simulink model "PUMA_Dynamicssoal4"  (R2026a)
settings: Solver=ode45  StopTime=15  EnableMultiTasking=on
settings Model: Creator=imi-pc
settings DataIOCC: SaveFormat=StructureWithTime
settings HardwareCC: ProdHWDeviceType=Specified
settings GRTTargetCC: CombineOutputUpdateFcns=off  GRTInterface=on

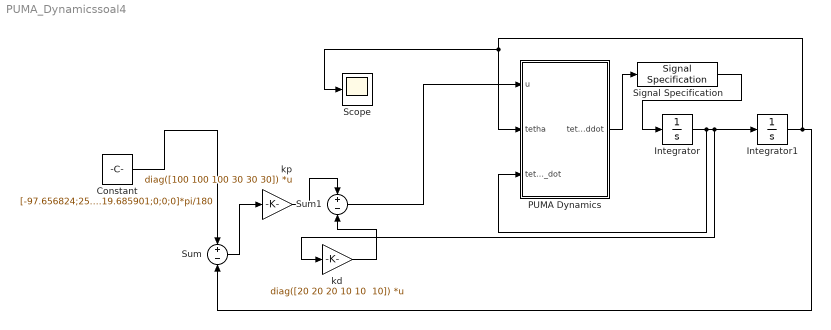
== system PUMA_Dynamicssoal4 ==
  Constant : Constant  Value=[-97.656824;25.988513;-19.685901;0;0;0]*pi/180
  Integrator : Integrator
  Integrator1 : Integrator
  PUMA Dynamics : MATLAB Function  TreatAsAtomicUnit=on
  Scope : Scope
      settings: ActiveDisplayYMinimum=-15.492496269263574  ActiveDisplayYMaximum=5.656821021719038
  Signal Specification : SignalSpecification  Dimensions=[6 1]
  Sum : Sum  Inputs=+-
  Sum1 : Sum  Inputs=+-
  kd : Gain  Gain="diag([20 20 20 10 10  10])"  Multiplication=Matrix(K*u)
  kp : Gain  Gain=diag([100 100 100 30 30 30])  Multiplication=Matrix(K*u)
  wires:
  Integrator/1 -> PUMA Dynamics/3(tetha_dot), kd/1, Integrator1/1
  Constant/1 -> Sum/1
  Sum/1 -> kp/1
  kd/1 -> Sum1/2
  kp/1 -> Sum1/1
  Sum1/1 -> PUMA Dynamics/1(u)
  PUMA Dynamics/1(tetha_ddot) -> Signal Specification/1
  Signal Specification/1 -> Integrator/1
  Integrator1/1 -> Scope/1, PUMA Dynamics/2(tetha), Sum/2

== matlab function PUMA_Dynamicssoal4/PUMA Dynamics ==
  data: u input; tetha input; tetha_ddot output; tetha_dot input
function tetha_ddot = fcn(u,tetha,tetha_dot)






c2=cos(tetha(2));
s2=sin(tetha(2));

c3=cos(tetha(3));
s3=sin(tetha(3));

c23=cos(tetha(2)+tetha(3));
s23=sin(tetha(2)+tetha(3));

c223=cos(2*tetha(2)+tetha(3));
s223=sin(2*tetha(2)+tetha(3));



%Inertial Constants (kg.m^2)
I1=1.43; %+-.05
I2=1.75;
I3=1.38;
I4=.69;
I5=.372;
I6=.333;
I7=.298;
I8=-.134;
I9=.0238;
I10=-.0213;
I11=-.0142;
I12=-.011;
I13=-.00379;
I14=.00164;
I15=.00125;
I16=.00124;
I17=.000642;
I18=.000431;
I19=.0003;
I20=-.000202;
I21=-.0001;
I22=-.000058;
I23=.00004;

Im1=1.14;
Im2=4.71;
Im3=.827;
Im4=.2;
Im5=.179;
Im6=.193;

%gravitational constants (N.m)
g1=-37.2;
g2=-8.44;
g3=1.02;
g4=.249;
g5=-.0282;

%here are the robot matrices A, B, C and G
% A matrix

a11=Im1+I1+I3*c2^2+I7*s23^2+I10*s23*c23+I11*s2*c2+I21*s23^2+2*(I5*c2*s23+I12*c2*c23+I15*s23*s23+I16*c2*s23+I22*s23*c23);
a12=I4*s2+I8*c23+I9*c2+I13*s23-I18*c23;
a13=I8*c23+I13*s23-I18*c23;

a22=Im2+I2+I6+2*(I5*s3+I12*c2+I15+I16*s3);
a23=I5*s3+I6+I12*c3+I16*s3+2*I15;

a33=Im3+I6+2*I15;
a35=I15+I17;

a44=Im4+I14;

a55=Im5+I17;

a66=Im6+I23;

a21=a12; a31=a13; a32=a23;

a14=0;
a15=0;
a16=0;

a24=0;
a25=0;
a26=0;

a34=0;
a36=0;

a41=0;
a42=0;
a43=0;
a45=0;
a46=0;

a51=0;
a52=0;
a53=0;
a54=0;
a56=0;

a61=0;
a62=0;
a63=0;
a64=0;
a65=0;


%and here is the A matrix
A= [a11 a12 a13 a14 a15 a16;
    a21 a22 a23 a24 a25 a26;
    a31 a32 a33 a34 a35 a36;
    a41 a42 a43 a44 a45 a46;
    a51 a52 a53 a54 a55 a56;
    a61 a62 a63 a64 a65 a66];





% B matrix
b112=2*(-I3*s2*c2+I5*c223+I7*s23*c23-I12*s223+I15*2*s23*c23+I16*c223+I21*s23*c23+I22*(1-2*s23^2))+I10*(1-2*s23^2)+I11*(1-2*s2^2);
b113=2*(I5*c23*c2+I7*s23*c23-I12*s23*c2+I15*2*s23*c23+I16*c2*c23+I21*s23*c23+I22*(1-2*s23^2))+I10*(1-2*s23^2);
b115=2*(-s23*c23+I15*s23*c23+I16*c2*c23+I22*c23^2);
b123=2*(-I8*s23+I13*c23+I18*s23);
b214=I14*s23+I19*s23+I20*s23;
b223=2*(-I12*s3+I5*c3+I16*c3);
b225=2*(I16*c3+I22);
b235=b225;
b314=(I20*+I14+I19)*s23;
b412=-b214;
b413=-b314;
b415=-I20*s23-I17*s23;
b514=-b415;


%and here is the B matrix
B= [b112 b113 0 b115 0 b123 0 0 0 0 0 0 0 0 0;
    0 0 b214 0 0 b223 0 b225 0 0 b235 0 0 0 0;
    0 0 b314 0 0 0 0 0 0 0 0 0 0 0 0;
    b412 b413 0 b415 0 0 0 0 0 0 0 0 0 0 0;
    0 0 b514 0 0 0 0 0 0 0 0 0 0 0 0;
    0 0 0 0 0 0 0 0 0 0 0 0 0 0 0;];



% matrix C
c12=I4*c2-I8*s23-I9*s2+I13*c23+I18*s23;
c13=.5*b123;
c21=-.5*b112;
c23=.5*b223;
c31=-.5*b113;
c32=-c23;
c51=-.5*b115;
c52=-.5*b225;


%and here is the C matrix
C= [0 c12 c13 0 0 0;
    c21 0 c23 0 0 0;
    c31 c32 0 0 0 0;
    0 0 0 0 0 0;
    c51 c52 0 0 0 0;
    0 0 0 0 0 0];




% G matrix
G2=g1*c2+g2*s23+g3*s2+g4*c23+g5*s23;
G3=g2*s23+g4*c23+g5*s23;
G5=g5*s23;


%here is vector G
G=[0;g2;g3;0;g5;0];

d_theta_t=[tetha_dot(1)*tetha_dot(2);tetha_dot(1)*tetha_dot(3);0;0;0;tetha_dot(2)*tetha_dot(3);0;0;0;0;0;0;0;0;0];
%%%%%%%%%%%%%%%%%%%%%%%%%%%%%%%%%%%%%

tetha_ddot=inv(A)*(u-B*d_theta_t-C*tetha_dot.^2-G);
